simulink model "My_gfm_battery_sil_x"  (R2018b)
settings: Solver=ode45  StartTime=0.0  StopTime=10  MaxStep=1e-4  RelTol=1e-3
PreLoadFcn:
  | modelDir = fileparts(get_param(bdroot,'FileName'));
  | 
  | load_system(fullfile(modelDir,'controls_element_lib.slx'));
  | load_system(fullfile(modelDir,'test_sequence_lib.slx'));
InitFcn:
  | close all;
  | clear all;
  | clc;
  | 
  | % frequency nominals
  | F_NOM = 60;
  | W_NOM = 2 * pi * F_NOM;
  | 
  | % base values relative to inverter
  | % --------------------------------
  | VLL_INV_NOM = 480;
  | P_INV_NOM = 1e6;
  | Q_INV_NOM = 0.5e6;
  | S_INV_NOM = sqrt(P_INV_NOM^2 + Q_INV_NOM^2);
  | 
  | I_INV_BASE = S_INV_NOM/(sqrt(3)*VLL_INV_NOM);
  | Z_INV_BASE = VLL_INV_NOM^2/S_INV_NOM;
  | L_INV_BASE = Z_INV_BASE / W_NOM;
  | C_INV_BASE = 1 / (Z_INV_BASE * W_NOM);
  | 
  | % nominal ratings for power system model
  | % --------------------------------------
  | INVERTER_COUNT = 100;
  | 
  | VLV_NOM = VLL_INV_NOM;
  | VMV_NOM = 35e3;
  | VHV_NOM = 230e3;
  | S_PLANT = INVERTER_COUNT * S_INV_NOM;
  | 
  | N_GSU = VHV_NOM/VMV_NOM;
  | N_MVT = VMV_NOM/VLV_NOM;
  | 
  | I_LV_BASE = S_PLANT/(sqrt(3)*VLV_NOM);
  | I_MV_BASE = S_PLANT/(sqrt(3)*VMV_NOM);
  | I_HV_BASE = S_PLANT/(sqrt(3)*VHV_NOM);
  | 
  | Z_LV_BASE = VLV_NOM^2/S_PLANT;
  | Z_MV_BASE = VMV_NOM^2/S_PLANT;
  | Z_HV_BASE = VHV_NOM^2/S_PLANT;
  | 
  | L_LV_BASE = Z_LV_BASE / W_NOM;
  | L_MV_BASE = Z_MV_BASE / W_NOM;
  | L_HV_BASE = Z_HV_BASE / W_NOM;
  | C_LV_BASE = 1 / (Z_LV_BASE * W_NOM);
  | C_MV_BASE = 1 / (Z_MV_BASE * W_NOM);
  | C_HV_BASE = 1 / (Z_HV_BASE * W_NOM);
undefined symbols (not defined in the file): j
libraries: controls_element_lib x19, simulink x19, test_sequence_lib x12
(part 1 of 4)
settings Model: SimulationMode=accelerator  Creator=HussamAlatrash  LastModifiedBy=ahhei
settings DataIOCC: ReturnWorkspaceOutputs=on
settings OptimizationCC: EfficientMapNaN2IntZero=off
settings DebuggingCC: UnconnectedInputMsg=none  UnconnectedOutputMsg=none  UnconnectedLineMsg=none
settings HardwareCC: TargetBitPerPointer=64  TargetBitPerSizeT=64  TargetBitPerPtrDiffT=64  TargetLongLongMode=on  TargetIntDivRoundTo=Zero  TargetEndianess=LittleEndian  TargetWordSize=64  TargetHWDeviceType=MATLAB Host  ProdEqTarget=off
settings ModelReferenceCC: EnableRefExpFcnMdlSchedulingChecks=off
settings CodeAppCC: MaxIdLength=128
settings GRTTargetCC: TargetLangStandard=C89/C90 (ANSI)  CombineOutputUpdateFcns=off  GRTInterface=on

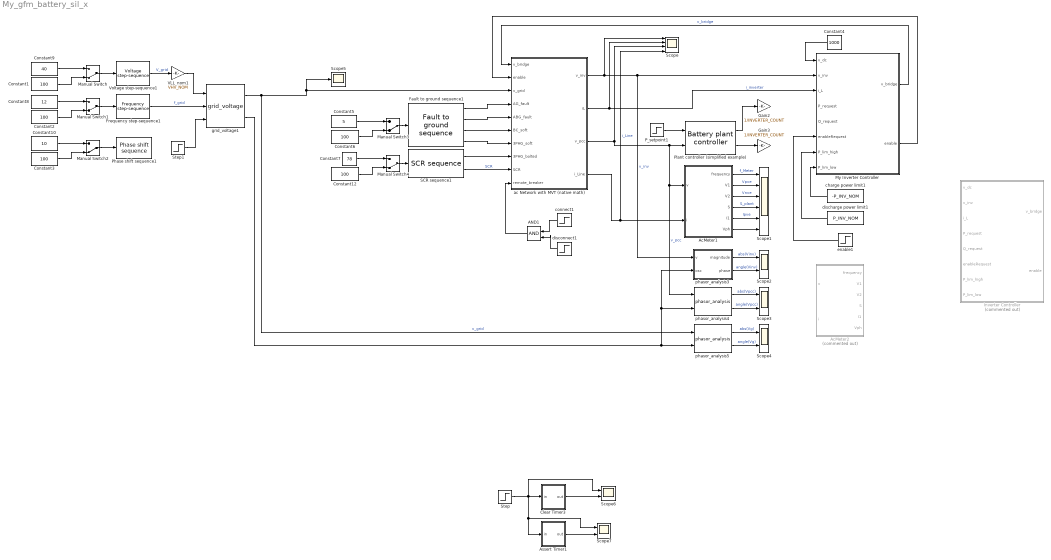
== system My_gfm_battery_sil_x ==
  " Inverter Controller" : Subsystem  Commented=on
  AND1 : Logic  IconShape=distinctive  AllPortsSameDT=off  OutDataTypeStr=boolean
  AcMeter1 : Subsystem  AncestorBlock=test_sequence_lib/AcMeter  mask{VllRated=VHV_NOM}
      mask prompts: VllRated "Rated line voltage"
  AcMeter2 : Subsystem  Commented=on  AncestorBlock=test_sequence_lib/AcMeter  mask{VllRated=VHV_NOM}
      mask prompts: VllRated "Rated line voltage"
  Assert Timer1 : Subsystem  mask{T_STEP=1e-3, TIMEOUT=3e-3}
      mask prompts: T_STEP "Time step"
  Clear Timer3 : Subsystem  mask{T_STEP=1e-3, TIMEOUT=3e-3, TIMER_INIT=0}
      mask prompts: T_STEP "Time step"; TIMER_INIT "Timer initial value"
  Constant{1..3,6,12} (5 alike) : Constant  Value=100
  Constant10 : Constant  Value=10
  Constant4 : Constant  Value=1000
  Constant5 : Constant  Value=5
  Constant7 : Constant  Value=78
  Constant8 : Constant  Value=12
  Constant9 : Constant  Value=40
  Fault to ground sequence1 : test_sequence_lib/Fault to ground sequence  SystemSampleTime=-1
  Frequency step-sequence1 : test_sequence_lib/Frequency step-sequence  SystemSampleTime=-1
  Gain2 : Gain  Gain=1/INVERTER_COUNT
  Gain3 : Gain  Gain=1/INVERTER_COUNT
  Manual Switch{,1..4} (5 alike) : ManualSwitch  CurrentSetting=0
  "My Inverter Controller " : Subsystem
  P_setpoint1 : Step  Time=4  After=S_PLANT*0.5  SampleTime=0
  Phase shift sequence1 : test_sequence_lib/Phase shift sequence  SystemSampleTime=-1
  Plant controller (simplified example) : controls_element_lib/Battery plant controller  SystemSampleTime=-1
  SCR sequence1 : test_sequence_lib/SCR sequence  SystemSampleTime=-1
  Scope : Scope  NumInputPorts=4
  Scope1 : Scope  NumInputPorts=6
  Scope{2..4,6..7} (5 alike) : Scope  NumInputPorts=2
  Scope5 : Scope
  Step : Step  Before=1  After=0  SampleTime=0
  Step1 : Step  Time=6  After=10*pi/180  SampleTime=0
  VLL_nom1 : Gain  Gain=VHV_NOM
  Voltage step-sequence1 : test_sequence_lib/Voltage step-sequence  SystemSampleTime=-1
  ac Network with MVT (native math) : Subsystem  AncestorBlock=test_sequence_lib/ac Network with MVT (native math)
  charge power limit1 : Constant  Value=-P_INV_NOM
  connect1 : Step  Time=0  SampleTime=0
  discharge power limit1 : Constant  Value=P_INV_NOM
  disconnect1 : Step  Time=10  Before=1  After=0  SampleTime=0
  enable1 : Step  Time=0.5  SampleTime=0
  grid_voltage1 : test_sequence_lib/grid_voltage  SystemSampleTime=-1
  phasor_analysis3 : Subsystem  AncestorBlock=test_sequence_lib/phasor_analysis
  phasor_analysis4 : test_sequence_lib/phasor_analysis  SystemSampleTime=-1
  phasor_analysis5 : test_sequence_lib/phasor_analysis  SystemSampleTime=-1
  wires:
  Voltage step-sequence1/1 -> VLL_nom1/1  "V_grid"
  Manual Switch/1 -> Voltage step-sequence1/1
  Fault to ground sequence1/2 -> ac Network with MVT (native math)/5(ABG_fault)
  AND1/1 -> ac Network with MVT (native math)/10(remote_breaker)
  Constant4/1 -> "My Inverter Controller "/1(v_dc)
  AcMeter1/3(V2) -> Scope1/3  "Vnve"
  discharge power limit1/1 -> "My Inverter Controller "/7(P_lim_high)
  Fault to ground sequence1/3 -> ac Network with MVT (native math)/6(BC_soft)
  AcMeter1/6(Vph) -> Scope1/6
  "My Inverter Controller "/1(v_bridge) -> ac Network with MVT (native math)/1(v_bridge)  "v_bridge"
  AcMeter1/2(V1) -> Scope1/2  "Vpve"
  Plant controller (simplified example)/1 -> Gain2/1
  ac Network with MVT (native math)/1(v_inv) -> phasor_analysis3/1(v), "My Inverter Controller "/2(v_inv), Scope/1  "v_inv"
  P_setpoint1/1 -> Plant controller (simplified example)/1
  phasor_analysis5/1 -> Scope4/1  "abs(Vg)"
  AcMeter1/5(I1) -> Scope1/5  "Ipve"
  Plant controller (simplified example)/2 -> Gain3/1
  grid_voltage1/1 -> phasor_analysis5/1, Scope5/1, ac Network with MVT (native math)/3(v_grid)  "v_grid"
  SCR sequence1/1 -> ac Network with MVT (native math)/8(3PHG_bolted)
  phasor_analysis3/1(magnitude) -> Scope2/1  "abs(Vinv)"
  AcMeter1/4(S) -> Scope1/4  "S_plant"
  ac Network with MVT (native math)/4(i_Line) -> Scope/4, AcMeter1/2(i)  "i_Line"
  AcMeter1/1(frequency) -> Scope1/1  "f_Meter"
  VLL_nom1/1 -> grid_voltage1/1
  phasor_analysis3/2(phase) -> Scope2/2  "angle(Vinv)"
  SCR sequence1/2 -> ac Network with MVT (native math)/9(SCR)  "SCR"
  ac Network with MVT (native math)/2(iL) -> "My Inverter Controller "/3(i_L), Scope/2  "i_inverter"
  disconnect1/1 -> AND1/2
  Fault to ground sequence1/4 -> ac Network with MVT (native math)/7(3PHG_soft)
  ac Network with MVT (native math)/3(v_pcc) -> Plant controller (simplified example)/2, phasor_analysis4/1, AcMeter1/1(v), Scope/3  "v_pcc"
  charge power limit1/1 -> "My Inverter Controller "/8(P_lim_low)
  "My Inverter Controller "/2(enable) -> ac Network with MVT (native math)/2(enable)
  Frequency step-sequence1/1 -> grid_voltage1/2  "f_grid"
  Fault to ground sequence1/1 -> ac Network with MVT (native math)/4(AG_fault)
  grid_voltage1/2 -> phasor_analysis4/2, phasor_analysis3/2(osc), phasor_analysis5/2
  phasor_analysis5/2 -> Scope4/2  "angle(Vg)"
  enable1/1 -> "My Inverter Controller "/6(enableRequest)
  connect1/1 -> AND1/1
  Constant9/1 -> Manual Switch/1
  Constant1/1 -> Manual Switch/2
  Constant2/1 -> Manual Switch1/2
  Manual Switch1/1 -> Frequency step-sequence1/1
  Constant8/1 -> Manual Switch1/1
  Manual Switch2/1 -> Phase shift sequence1/1
  Constant3/1 -> Manual Switch2/2
  Constant10/1 -> Manual Switch2/1
  Constant6/1 -> Manual Switch3/2
  Constant5/1 -> Manual Switch3/1
  Manual Switch3/1 -> Fault to ground sequence1/1
  Constant7/1 -> Manual Switch4/1
  Constant12/1 -> Manual Switch4/2
  Manual Switch4/1 -> SCR sequence1/1
  phasor_analysis4/1 -> Scope3/1  "abs(Vpcc)"
  phasor_analysis4/2 -> Scope3/2  "angle(Vpcc)"
  Step/1 -> Scope7/1, Assert Timer1/1(in), Scope6/1, Clear Timer3/1(in)
  Clear Timer3/1(out) -> Scope6/2
  Assert Timer1/1(out) -> Scope7/2
  Step1/1 -> grid_voltage1/3

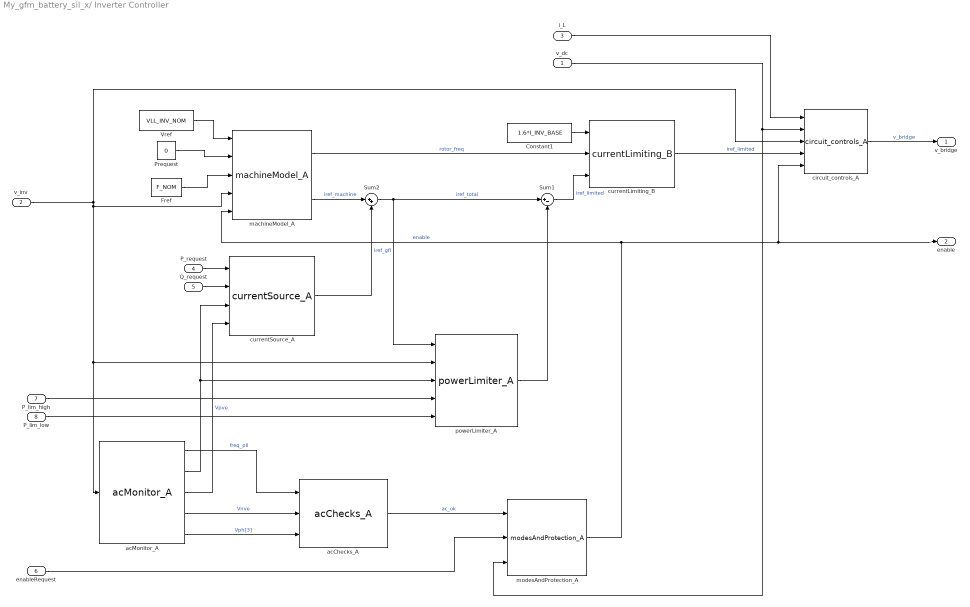
== system My_gfm_battery_sil_x/ Inverter Controller ==
  v_dc : Inport
  v_inv : Inport  Port=2
  i_L : Inport  Port=3
  P_request : Inport  Port=4
  Q_request : Inport  Port=5
  enableRequest : Inport  Port=6
  P_lim_high : Inport  Port=7
  P_lim_low : Inport  Port=8
  Constant1 : Constant  Value=1.6*I_INV_BASE
  Fref : Constant  Value=F_NOM
  Prequest : Constant  Value=0
  Sum1 : Sum  Inputs=|+-
  Sum2 : Sum  Inputs=|++
  Vref : Constant  Value=VLL_INV_NOM
  acChecks_A : controls_element_lib/acChecks_A  VllRated=VLL_INV_NOM  nominalFrequency=F_NOM  tRequalify=2  T_CNTL=1e-3
  "acMonitor_A " : controls_element_lib/acMonitor_A  VllRated=VLL_INV_NOM  nominalFrequency=F_NOM
  circuit_controls_A : controls_element_lib/circuit_controls_A  SystemSampleTime=-1
  currentLimiting_B : controls_element_lib/currentLimiting_B  IRated=I_INV_BASE  peakSoftLimit=2.6  peakHardLimit=3.6
  currentSource_A : controls_element_lib/currentSource_A  VllRated=VLL_INV_NOM  SRated=S_INV_NOM  nominalFrequency=F_NOM  Plimit=P_INV_NOM/S_INV_NOM  Qlimit=Q_INV_NOM/S_INV_NOM
  machineModel_A : controls_element_lib/machineModel_A  SRated=S_INV_NOM  VllRated=VLL_INV_NOM  nominalFrequency=F_NOM  inertialConstant=2.5  kDroop=1  kDamper=2  Xs=0.3  rs=0.08  Qlimit=0.5  wExciter=10
  modesAndProtection_A : controls_element_lib/modesAndProtection_A  dcOvervotlageThreshold=1800  dcUndervotlageThreshold=700  dcTripClearTimeout=0.2
  powerLimiter_A : controls_element_lib/powerLimiter_A  VllRated=VLL_INV_NOM  nominalFrequency=F_NOM  wPowerLimiter=3
  v_bridge : Outport  VectorParamsAs1DForOutWhenUnconnected=on
  enable : Outport  Port=2  VectorParamsAs1DForOutWhenUnconnected=on
  wires:
  Vref/1 -> machineModel_A/1
  Prequest/1 -> machineModel_A/2
  Fref/1 -> machineModel_A/3
  machineModel_A/2 -> Sum2/1  "iref_machine"
  "acMonitor_A "/2 -> currentSource_A/3, powerLimiter_A/3
  Sum1/1 -> currentLimiting_B/3  "iref_limited"
  currentSource_A/1 -> Sum2/2  "iref_gfl"
  Sum2/1 -> Sum1/1, powerLimiter_A/1  "iref_total"
  "acMonitor_A "/3 -> currentSource_A/4  "Vpve"
  Q_request/1 -> currentSource_A/2
  P_request/1 -> currentSource_A/1
  enableRequest/1 -> modesAndProtection_A/2
  modesAndProtection_A/1 -> circuit_controls_A/5, enable/1, machineModel_A/5  "enable"
  "acMonitor_A "/5 -> acChecks_A/3  "Vph[3]"
  acChecks_A/1 -> modesAndProtection_A/1  "ac_ok"
  Constant1/1 -> currentLimiting_B/1
  "acMonitor_A "/1 -> acChecks_A/1  "freq_pll"
  "acMonitor_A "/4 -> acChecks_A/2  "Vnve"
  P_lim_low/1 -> powerLimiter_A/5
  P_lim_high/1 -> powerLimiter_A/4
  powerLimiter_A/1 -> Sum1/2
  v_dc/1 -> circuit_controls_A/2, modesAndProtection_A/3
  circuit_controls_A/1 -> v_bridge/1  "v_bridge"
  machineModel_A/1 -> currentLimiting_B/2  "rotor_freq"
  i_L/1 -> circuit_controls_A/1
  v_inv/1 -> "acMonitor_A "/1, powerLimiter_A/2, machineModel_A/4, circuit_controls_A/3
  currentLimiting_B/1 -> circuit_controls_A/4  "iref_limited"

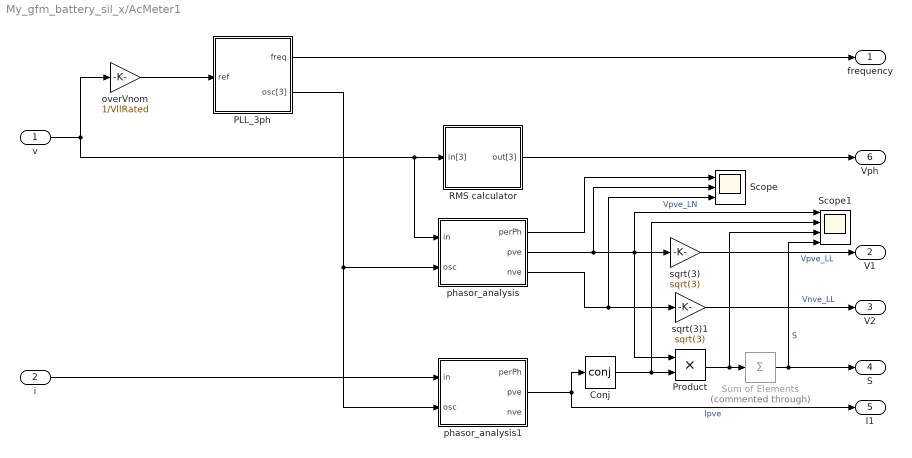
== system My_gfm_battery_sil_x/AcMeter1 ==
  v : Inport
  i : Inport  Port=2
  Conj : Math  Operator=conj  SaturateOnIntegerOverflow=on
  PLL_3ph : Subsystem
  Product : Product
  RMS calculator : Subsystem
  Scope : Scope  NumInputPorts=3
  Scope1 : Scope  NumInputPorts=4
  Sum of Elements : Sum  Commented=through  Inputs=+
  overVnom : Gain  Gain=1/VllRated
  phasor_analysis : Subsystem
  phasor_analysis1 : Subsystem  AncestorBlock=test_sequence_lib/AcMeter/phasor_analysis
  sqrt(3) : Gain  Gain=sqrt(3)
  sqrt(3)1 : Gain  Gain=sqrt(3)
  frequency : Outport  VectorParamsAs1DForOutWhenUnconnected=on
  V1 : Outport  Port=2  VectorParamsAs1DForOutWhenUnconnected=on
  V2 : Outport  Port=3  VectorParamsAs1DForOutWhenUnconnected=on
  S : Outport  Port=4  VectorParamsAs1DForOutWhenUnconnected=on
  I1 : Outport  Port=5  VectorParamsAs1DForOutWhenUnconnected=on
  Vph : Outport  Port=6  VectorParamsAs1DForOutWhenUnconnected=on
  wires:
  RMS calculator/1(out[3]) -> Vph/1
  PLL_3ph/2(osc[3]) -> phasor_analysis/2(osc), phasor_analysis1/2(osc)
  phasor_analysis/1(perPh) -> Scope/1
  Sum of Elements/1 -> Scope1/4, S/1  "S"
  v/1 -> RMS calculator/1(in[3]), phasor_analysis/1(in), overVnom/1
  PLL_3ph/1(freq) -> frequency/1
  overVnom/1 -> PLL_3ph/1(ref)
  Conj/1 -> Scope1/2, Product/2
  Product/1 -> Scope1/3, Sum of Elements/1
  phasor_analysis/2(pve) -> Scope/2, Scope1/1, Product/1, sqrt(3)/1  "Vpve_LN"
  phasor_analysis/3(nve) -> Scope/3, sqrt(3)1/1
  phasor_analysis1/2(pve) -> I1/1, Conj/1  "Ipve"
  sqrt(3)1/1 -> V2/1  "Vnve_LL"
  i/1 -> phasor_analysis1/1(in)
  sqrt(3)/1 -> V1/1  "Vpve_LL"

== system My_gfm_battery_sil_x/AcMeter2 ==
  v : Inport
  i : Inport  Port=2
  Conj : Math  Operator=conj  SaturateOnIntegerOverflow=on
  PLL_3ph : Subsystem
  Product : Product
  RMS calculator : Subsystem
  Scope : Scope  NumInputPorts=3
  Scope1 : Scope  NumInputPorts=4
  Sum of Elements : Sum  Inputs=+
  overVnom : Gain  Gain=1/VllRated
  phasor_analysis : Subsystem
  phasor_analysis1 : Subsystem  AncestorBlock=test_sequence_lib/AcMeter/phasor_analysis
  sqrt(3) : Gain  Gain=sqrt(3)
  sqrt(3)1 : Gain  Gain=sqrt(3)
  frequency : Outport  VectorParamsAs1DForOutWhenUnconnected=on
  V1 : Outport  Port=2  VectorParamsAs1DForOutWhenUnconnected=on
  V2 : Outport  Port=3  VectorParamsAs1DForOutWhenUnconnected=on
  S : Outport  Port=4  VectorParamsAs1DForOutWhenUnconnected=on
  I1 : Outport  Port=5  VectorParamsAs1DForOutWhenUnconnected=on
  Vph : Outport  Port=6  VectorParamsAs1DForOutWhenUnconnected=on
  wires:
  RMS calculator/1(out[3]) -> Vph/1
  PLL_3ph/2(osc[3]) -> phasor_analysis/2(osc), phasor_analysis1/2(osc)
  phasor_analysis/1(perPh) -> Scope/1, Product/1, Scope1/1
  Sum of Elements/1 -> Scope1/4, S/1  "S"
  v/1 -> RMS calculator/1(in[3]), phasor_analysis/1(in), overVnom/1
  PLL_3ph/1(freq) -> frequency/1
  phasor_analysis1/1(perPh) -> Conj/1
  overVnom/1 -> PLL_3ph/1(ref)
  Conj/1 -> Scope1/2, Product/2
  Product/1 -> Scope1/3, Sum of Elements/1
  phasor_analysis/2(pve) -> Scope/2, sqrt(3)/1  "Vpve_LN"
  phasor_analysis/3(nve) -> Scope/3, sqrt(3)1/1
  phasor_analysis1/2(pve) -> I1/1  "Ipve"
  sqrt(3)1/1 -> V2/1  "Vnve_LL"
  i/1 -> phasor_analysis1/1(in)
  sqrt(3)/1 -> V1/1  "Vpve_LL"

== system My_gfm_battery_sil_x/Assert Timer1 ==
  in : Inport
  Constant : Constant  Value=T_STEP
  Constant1 : Constant  Value=0
  Constant2 : Constant  Value=TIMEOUT
  Constant3 : Constant  Value=T_STEP
  Gain : Gain  Gain=0
  Min1 : MinMax  Function=max  Inputs=2
  Min2 : MinMax  Inputs=2
  Relational Operator : RelationalOperator  Operator=>  OutDataTypeStr=boolean  RndMeth=Simplest
  Sum1 : Sum  Inputs=|++
  Sum2 : Sum  Inputs=|++
  Switch : Switch  Criteria=u2 > Threshold
  Unit Delay : UnitDelay  SampleTime=T_STEP
  out : Outport  VectorParamsAs1DForOutWhenUnconnected=on
  wires:
  Sum2/1 -> Relational Operator/1, Min2/1
  Sum1/1 -> Min2/2, Relational Operator/2
  Constant/1 -> Sum2/1
  Min2/1 -> Switch/1
  Constant1/1 -> Switch/3
  Unit Delay/1 -> Sum2/2
  in/1 -> Switch/2
  Switch/1 -> Unit Delay/1
  Relational Operator/1 -> out/1
  Min1/1 -> Sum1/1
  Constant2/1 -> Min1/1
  Constant3/1 -> Min1/2, Gain/1
  Gain/1 -> Sum1/2

== system My_gfm_battery_sil_x/Clear Timer3 ==
  note: One sample delay on Rise
  in : Inport
  Constant : Constant  Value=T_STEP
  Constant1 : Constant  Value=0
  Constant2 : Constant  Value=TIMEOUT
  Constant3 : Constant  Value=T_STEP
  Min1 : MinMax  Function=max  Inputs=2
  Min2 : MinMax  Function=max  Inputs=2
  Relational Operator : RelationalOperator  Operator=>  OutDataTypeStr=boolean  RndMeth=Simplest
  Sum1 : Sum  Inputs=|++
  Sum2 : Sum  Inputs=|-+
  Switch : Switch  Criteria=u2 > Threshold
  Unit Delay : UnitDelay  InitialCondition=TIMER_INIT  SampleTime=T_STEP
  out : Outport  VectorParamsAs1DForOutWhenUnconnected=on
  wires:
  Sum1/1 -> Switch/1
  Sum2/1 -> Relational Operator/1, Min2/1
  Constant/1 -> Sum2/1
  Min2/1 -> Switch/3
  Constant1/1 -> Min2/2, Relational Operator/2
  Unit Delay/1 -> Sum2/2
  in/1 -> Switch/2
  Switch/1 -> Unit Delay/1
  Relational Operator/1 -> out/1
  Constant2/1 -> Min1/1
  Constant3/1 -> Min1/2, Sum1/2
  Min1/1 -> Sum1/1

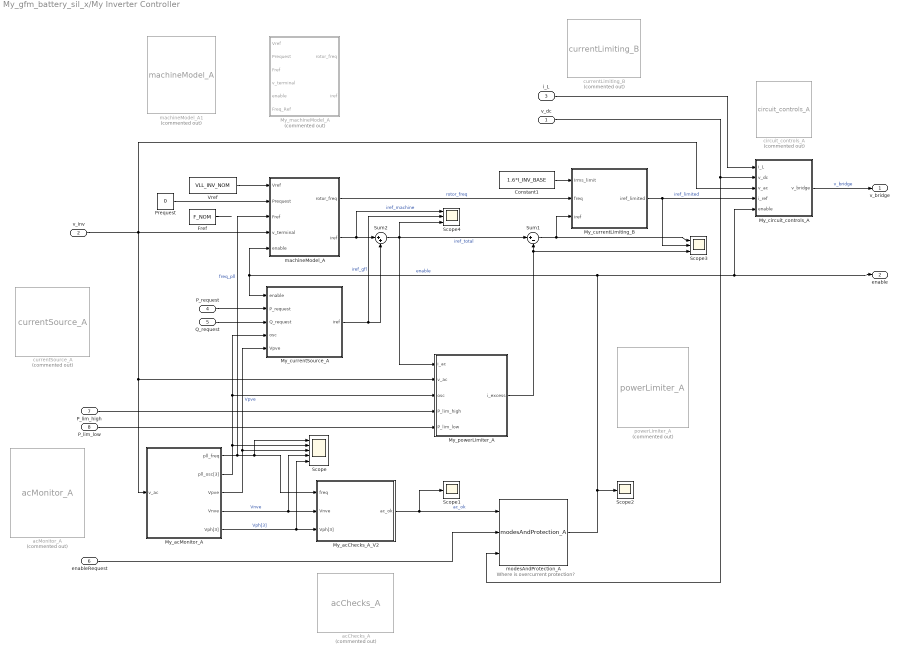
== system My_gfm_battery_sil_x/My Inverter Controller  ==
  note: Where is overcurrent protection?
  v_dc : Inport
  v_inv : Inport  Port=2
  i_L : Inport  Port=3
  P_request : Inport  Port=4
  Q_request : Inport  Port=5
  enableRequest : Inport  Port=6
  P_lim_high : Inport  Port=7
  P_lim_low : Inport  Port=8
  Constant1 : Constant  Value=1.6*I_INV_BASE
  Fref : Constant  Value=F_NOM
  My_acChecks_A_V2 : Subsystem  AncestorBlock=controls_element_lib/acChecks_A  mask{VllRated=VLL_INV_NOM, NominalFrequency=F_NOM, Ts=1e-3, Time1=2, Time2=0, VHi=1.15, VLo=0.85, FHi=62, FLo=58, VNeg=0.2, Time3=0, OV3=1.3, OV3_Time=0.02, OV3_en=1, OV2=1.25, OV2_Time=2, OV2_en=1, OV1=1.2, OV1_Time=20, OV1_en=1, UV1=0.81, UV1_Time=15, UV1_en=1, UV2=0.5, UV2_Time=5, UV2_en=1, UV3=0.2, UV3_Time=1, UV3_en=1, OF3=70, OF3_Time=0.2, OF3_en=1, OF2=65, OF2_Time=10, OF2_en=1, OF1=63, OF1_Time=30, OF1_en=1, UF1=56, UF1_Time=30, UF1_en=1, UF2=55, UF2_Time=10, UF2_en=1, UF3=50, UF3_Time=0.2, UF3_en=1}
      mask prompts: VllRated "Rated Line-to-Line Voltage (V)"; NominalFrequency "Nominal Line Frequency (Hz)"; Ts "Operating Sample Time (sec)"; Time1 "Connection Time (sec)"; Time2 "Connection Out-of-Condition Delay (sec)"; VHi "High Voltage Threshold (pu)"; VLo "Low Voltage Threshold (pu)"; FHi "High Frequency Threshold (Hz)"; FLo "Low Frequency Threshold (Hz)"; VNeg "Negative Sequence Voltage Threshold (pu)"; Time3 "Trip Out-of-Condition Delay (sec)"; OV3 "OV PickUp 3 (pu)"; OV3_Time "OV Time 3 (sec)"; OV3_en "OV Enable 3"; OV2 "OV PickUp 2 (pu)"; OV2_Time "OV Time 2 (sec)"; OV2_en "OV Enable 2"; OV1 "OV PickUp 1 (pu)"; OV1_Time "OV Time 1 (sec)"; OV1_en "OV Enable 1"; UV1 "UV PickUp 1 (pu)"; UV1_Time "UV Time 1 (sec)"; UV1_en "UV Enable 1"; UV2 "UV PickUp 2 (pu)"; UV2_Time "UV Time 2 (sec)"; UV2_en "UV Enable 2"; UV3 "UV PickUp 3 (pu)"; UV3_Time "UV Time 3 (sec)"; UV3_en "UV Enable 3"; OF3 "OF PickUp 3 (Hz)"; OF3_Time "OF Time 3 (pu)"; OF3_en "OF Enable 3"; OF2 "OF PickUp 2 (Hz)"; OF2_Time "OF Time 2 (pu)"; OF2_en "OF Enable 2"; OF1 "OF PickUp 1 (Hz)"; OF1_Time "OF Time 1 (pu)"; OF1_en "OF Enable 1"; UF1 "UF PickUp 1 (Hz)"; UF1_Time "UF Time 1 (sec)"; UF1_en "UF Enable 1"; UF2 "UF PickUp 2 (Hz)"; UF2_Time "UF Time 2 (sec)"; UF2_en "UF Enable 2"; UF3 "UF PickUp 3 (Hz)"; UF3_Time "UF Time 3 (sec)"; UF3_en "UF Enable 3"
      mask DialogControl DescGroupVar Prompt: ACChecks
      mask DialogControl DecsTextVar Prompt: Grid Checks for Connection and Tripping
      mask DialogControl ParameterGroupVar Prompt: General Parameters
      mask DialogControl Container11 Prompt: Connection Settings
      mask DialogControl Container20 Prompt: Thresholds
      mask DialogControl Container3 Prompt: Trip Settings
      mask DialogControl Container12 Prompt: General Parameters
      mask DialogControl Container15 Prompt: Over Voltage Settings
      mask DialogControl Container4 Prompt: Over Voltage
      mask DialogControl Container19 Prompt: Under Voltage Settings
      mask DialogControl Container7 Prompt: Under Voltage
      mask DialogControl Container17 Prompt: Over Frequency Settings
      mask DialogControl Container9 Prompt: Over Frequency
      mask DialogControl Container16 Prompt: Under Frequency Settings
      mask DialogControl Container10 Prompt: Under Frequency
  My_acMonitor_A : Subsystem  AncestorBlock=controls_element_lib/acMonitor_A  mask{VllRated=VLL_INV_NOM, nominalFrequency=F_NOM}
      mask prompts: VllRated "Rated line-to-line voltage (V)"; nominalFrequency "Nominal line frequency (Hz)"
  My_circuit_controls_A : Subsystem  AncestorBlock=controls_element_lib/circuit_controls_A
  My_currentLimiting_B : Subsystem  AncestorBlock=controls_element_lib/currentLimiting_B  mask{IRated=I_INV_BASE, peakSoftLimit=2.6, peakHardLimit=3.6}
      mask prompts: IRated "Rated current (A)"; peakSoftLimit "Soft peak limit (pu)"; peakHardLimit "Hard peak limit (pu)"
  My_currentSource_A : Subsystem  AncestorBlock=controls_element_lib/currentSource_A  mask{VllRated=VLL_INV_NOM, SRated=S_INV_NOM, nominalFrequency=F_NOM, Plimit=P_INV_NOM/S_INV_NOM, Qlimit=Q_INV_NOM/S_INV_NOM}
      mask prompts: VllRated "Rated line-to-line voltage (V)"; SRated "Rated power (VA)"; nominalFrequency "Nominal line frequency (Hz)"; Plimit "Real power request limit (pu)"; Qlimit "Reactive power request limit (pu)"
  My_machineModel_A : Subsystem  Commented=on  AncestorBlock=controls_element_lib/machineModel_A  mask{SRated=S_INV_NOM, VllRated=VLL_INV_NOM, nominalFrequency=F_NOM, inertialConstant=2.5, kDroop=1, kDamper=2, Xs=0.3, rs=0.08, Qlimit=0.5, wExciter=10, FreqFF_Sel=0}
      mask prompts: SRated "Rated power (VA)"; VllRated "Rated Voltage (Volts, line-to-line)"; nominalFrequency "Nominal frequency (Hz)"; inertialConstant "Inertial constant (seconds)"; kDroop "Droop gain (pu/Hz)"; kDamper "Damper gain (pu/Hz)"; Xs "Stator reactance (pu)"; rs "Stator resistance (pu)"; Qlimit "Reactive power request limit (pu)"; wExciter "Exciter Bandwidth (rad)"; FreqFF_Sel "Frequency Feedforward Selector"
  My_powerLimiter_A : Subsystem  AncestorBlock=controls_element_lib/powerLimiter_A  mask{VllRated=VLL_INV_NOM, nominalFrequency=F_NOM, wPowerLimiter=3}
      mask prompts: VllRated "Rated line-to-line voltage (V)"; nominalFrequency "Nominal line frequency (Hz)"; wPowerLimiter "Bandwidth (rad)"
  Prequest : Constant  Value=0
  Scope : Scope  NumInputPorts=5
  Scope1 : Scope
  Scope2 : Scope
  Scope3 : Scope  NumInputPorts=3
  Scope4 : Scope  NumInputPorts=3
  Sum1 : Sum  Inputs=|+-
  Sum2 : Sum  Inputs=|++
  Vref : Constant  Value=VLL_INV_NOM
  acChecks_A : controls_element_lib/acChecks_A  Commented=on  VllRated=VLL_INV_NOM  nominalFrequency=F_NOM  tRequalify=2  T_CNTL=1e-3
  acMonitor_A : controls_element_lib/acMonitor_A  Commented=on  VllRated=VLL_INV_NOM  nominalFrequency=F_NOM
  circuit_controls_A : controls_element_lib/circuit_controls_A  Commented=on  SystemSampleTime=-1
  currentLimiting_B : controls_element_lib/currentLimiting_B  Commented=on  IRated=I_INV_BASE  peakSoftLimit=2.6  peakHardLimit=3.6
  currentSource_A : controls_element_lib/currentSource_A  Commented=on  VllRated=VLL_INV_NOM  SRated=S_INV_NOM  nominalFrequency=F_NOM  Plimit=P_INV_NOM/S_INV_NOM  Qlimit=Q_INV_NOM/S_INV_NOM
  machineModel_A : Subsystem  AncestorBlock=controls_element_lib/machineModel_A  mask{SRated=S_INV_NOM, VllRated=VLL_INV_NOM, nominalFrequency=F_NOM, inertialConstant=2.5, kDroop=1, kDamper=2, Xs=0.3, rs=0.08, Qlimit=0.5, wExciter=10}
      mask prompts: SRated "Rated power (VA)"; VllRated "Rated Voltage (Volts, line-to-line)"; nominalFrequency "Nominal frequency (Hz)"; inertialConstant "Inertial constant (seconds)"; kDroop "Droop gain (pu/Hz)"; kDamper "Damper gain (pu/Hz)"; Xs "Stator reactance (pu)"; rs "Stator resistance (pu)"; Qlimit "Reactive power request limit (pu)"; wExciter "Exciter Bandwidth (rad)"
  machineModel_A1 : controls_element_lib/machineModel_A  Commented=on  SRated=S_INV_NOM  VllRated=VLL_INV_NOM  nominalFrequency=F_NOM  inertialConstant=2.5  kDroop=1  kDamper=2  Xs=0.3  rs=0.08  Qlimit=0.5  wExciter=10
  modesAndProtection_A : controls_element_lib/modesAndProtection_A  dcOvervotlageThreshold=1800  dcUndervotlageThreshold=700  dcTripClearTimeout=0.2
  powerLimiter_A : controls_element_lib/powerLimiter_A  Commented=on  VllRated=VLL_INV_NOM  nominalFrequency=F_NOM  wPowerLimiter=3
  v_bridge : Outport  VectorParamsAs1DForOutWhenUnconnected=on
  enable : Outport  Port=2  VectorParamsAs1DForOutWhenUnconnected=on
  wires:
  Vref/1 -> machineModel_A/1(Vref)
  Prequest/1 -> machineModel_A/2(Prequest)
  machineModel_A/2(iref) -> Scope4/1, Sum2/1  "iref_machine"
  My_acMonitor_A/2(pll_osc[3]) -> Scope/2, My_currentSource_A/4(osc), My_powerLimiter_A/3(osc)
  My_currentLimiting_B/1(iref_limited) -> My_circuit_controls_A/4(i_ref), Scope3/2  "iref_limited"
  My_currentSource_A/1(iref) -> Sum2/2, Scope4/2  "iref_gfl"
  Sum2/1 -> Sum1/1, Scope4/3, My_powerLimiter_A/1(i_ac)  "iref_total"
  My_acMonitor_A/3(Vpve) -> My_currentSource_A/5(Vpve), Scope/3  "Vpve"
  Q_request/1 -> My_currentSource_A/3(Q_request)
  P_request/1 -> My_currentSource_A/2(P_request)
  enableRequest/1 -> modesAndProtection_A/2
  modesAndProtection_A/1 -> Scope2/1, machineModel_A/5(enable), My_currentSource_A/1(enable), My_circuit_controls_A/5(enable), enable/1  "enable"
  My_acMonitor_A/5(Vph[3]) -> My_acChecks_A_V2/3(Vph[3]), Scope/5  "Vph[3]"
  My_acChecks_A_V2/1(ac_ok) -> Scope1/1, modesAndProtection_A/1  "ac_ok"
  Constant1/1 -> My_currentLimiting_B/1(Irms_limit)
  My_acMonitor_A/1(pll_freq) -> machineModel_A/3(Fref), My_acChecks_A_V2/1(freq), Scope/1  "freq_pll"
  My_acMonitor_A/4(Vnve) -> My_acChecks_A_V2/2(Vnve), Scope/4  "Vnve"
  P_lim_low/1 -> My_powerLimiter_A/5(P_lim_low)
  P_lim_high/1 -> My_powerLimiter_A/4(P_lim_high)
  My_powerLimiter_A/1(i_excess) -> Sum1/2, Scope3/3
  Sum1/1 -> My_currentLimiting_B/3(iref), Scope3/1
  v_dc/1 -> My_circuit_controls_A/2(v_dc), modesAndProtection_A/3
  My_circuit_controls_A/1(v_bridge) -> v_bridge/1  "v_bridge"
  machineModel_A/1(rotor_freq) -> My_currentLimiting_B/2(freq)  "rotor_freq"
  i_L/1 -> My_circuit_controls_A/1(i_L)
  v_inv/1 -> My_acMonitor_A/1(v_ac), My_powerLimiter_A/2(v_ac), machineModel_A/4(v_terminal), My_circuit_controls_A/3(v_ac)
  Fref/1 -> ?

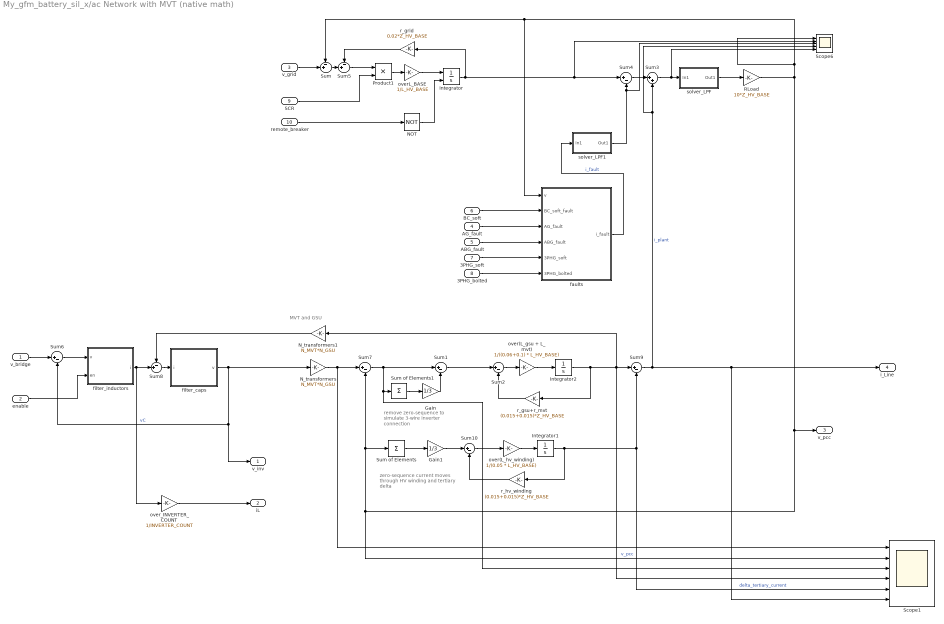
== system My_gfm_battery_sil_x/ac Network with MVT (native math) ==
  note: zero-sequence current moves through HV winding and tertiary delta
  note: remove zero-sequence to simulate 3-wire inverter connection
  note: MVT and GSU
  v_bridge : Inport
  enable : Inport  Port=2
  v_grid : Inport  Port=3
  AG_fault : Inport  Port=4
  ABG_fault : Inport  Port=5
  BC_soft : Inport  Port=6
  3PHG_soft : Inport  Port=7
  3PHG_bolted : Inport  Port=8
  SCR : Inport  Port=9
  remote_breaker : Inport  Port=10
  Gain : Gain  Gain=1/3
  Gain1 : Gain  Gain=1/3
  Integrator : Integrator  ExternalReset=level
  Integrator1 : Integrator
  Integrator2 : Integrator
  NOT : Logic  Operator=NOT  IconShape=distinctive  AllPortsSameDT=off  OutDataTypeStr=boolean
  N_transformers : Gain  Gain=N_MVT*N_GSU
  N_transformers1 : Gain  Gain=N_MVT*N_GSU
  Product1 : Product
  RLoad : Gain  Gain=10*Z_HV_BASE
  Scope1 : Scope  NumInputPorts=6
  Scope6 : Scope  NumInputPorts=5
  Sum : Sum  Inputs=-+|
  Sum of Elements : Sum  Inputs=+
  Sum of Elements1 : Sum  Inputs=+
  Sum{1..2,4,6..7,9..10} (7 alike) : Sum  Inputs=|+-
  Sum3 : Sum  Inputs=|++
  Sum5 : Sum  Inputs=-+|
  Sum8 : Sum  Inputs=-+|
  faults : Subsystem
  filter_caps : Subsystem
  filter_inductors : Subsystem
  over(L_gsu + L_mvt) : Gain  Gain=1/((0.06+0.1) * L_HV_BASE)
  over(L_hv_winding) : Gain  Gain=1/(0.05 * L_HV_BASE)
  overL_BASE : Gain  Gain=1/L_HV_BASE
  over_INVERTER_COUNT : Gain  Gain=1/INVERTER_COUNT
  r_grid : Gain  Gain=0.02*Z_HV_BASE
  r_gsu+r_mvt : Gain  Gain=(0.015+0.015)*Z_HV_BASE
  r_hv_winding : Gain  Gain=(0.015+0.015)*Z_HV_BASE
  solver_LPF : Subsystem
  solver_LPF1 : Subsystem
  v_inv : Outport  VectorParamsAs1DForOutWhenUnconnected=on
  iL : Outport  Port=2  VectorParamsAs1DForOutWhenUnconnected=on
  v_pcc : Outport  Port=3  VectorParamsAs1DForOutWhenUnconnected=on
  i_Line : Outport  Port=4  VectorParamsAs1DForOutWhenUnconnected=on
  wires:
  AG_fault/1 -> faults/3(AG_fault)
  ABG_fault/1 -> faults/4(ABG_fault)
  BC_soft/1 -> faults/2(BC_soft_fault)
  Gain1/1 -> Sum10/1
  Sum of Elements/1 -> Gain1/1
  Sum10/1 -> over(L_hv_winding)/1
  r_hv_winding/1 -> Sum10/2
  Integrator1/1 -> r_hv_winding/1, Scope1/5, Sum9/2  "delta_tertiary_current"
  over(L_hv_winding)/1 -> Integrator1/1
  Sum9/1 -> Scope1/6, i_Line/1, Scope6/4, Sum3/2  "i_plant"
  N_transformers1/1 -> Sum8/1
  N_transformers/1 -> Scope1/1, Sum7/1
  over_INVERTER_COUNT/1 -> iL/1
  filter_caps/1(v) -> N_transformers/1, Sum6/2, v_inv/1  "vC"
  Sum8/1 -> filter_caps/1(i)
  filter_inductors/1(i) -> over_INVERTER_COUNT/1, Sum8/2
  enable/1 -> filter_inductors/2(en)
  Sum6/1 -> filter_inductors/1(v)
  r_gsu+r_mvt/1 -> Sum2/2
  Sum1/1 -> Sum2/1
  Gain/1 -> Sum1/2
  Sum of Elements1/1 -> Gain/1
  Sum2/1 -> over(L_gsu + L_mvt)/1
  Sum7/1 -> Sum1/1, Scope1/3, Sum of Elements1/1
  over(L_gsu + L_mvt)/1 -> Integrator2/1
  solver_LPF/1(Out1) -> RLoad/1
  remote_breaker/1 -> NOT/1
  overL_BASE/1 -> Integrator/1
  Integrator/1 -> Scope6/2, Sum4/1, r_grid/1
  solver_LPF1/1(Out1) -> Scope6/3, Sum4/2
  RLoad/1 -> Sum of Elements/1, Sum7/2, Scope1/2, v_pcc/1, Sum/1, faults/1(v), Scope6/1  "v_pcc"
  faults/1(i_fault) -> solver_LPF1/1(In1)  "i_fault"
  3PHG_bolted/1 -> faults/6(3PHG_bolted)
  v_bridge/1 -> Sum6/1
  Product1/1 -> overL_BASE/1
  SCR/1 -> Product1/2
  r_grid/1 -> Sum5/1
  Sum3/1 -> Scope6/5, solver_LPF/1(In1)
  NOT/1 -> Integrator/2
  Sum4/1 -> Sum3/1
  v_grid/1 -> Sum/2
  Sum5/1 -> Product1/1
  Sum/1 -> Sum5/2
  Integrator2/1 -> Scope1/4, Sum9/1, N_transformers1/1, r_gsu+r_mvt/1
  3PHG_soft/1 -> faults/5(3PHG_soft)

== system My_gfm_battery_sil_x/phasor_analysis3 ==
  v : Inport
  osc : Inport  Port=2
  Complex to Magnitude-Angle : ComplexToMagnitudeAngle
  Complex to Real-Imag : ComplexToRealImag
  Conj : Math  Operator=conj  SaturateOnIntegerOverflow=on
  Gain : Gain  Gain=sqrt(2)
  Gain1 : Gain  Gain=1/3
  Gain2 : Gain  Gain=sqrt(3)
  Product3 : Product
  Real-Imag to Complex : RealImagToComplex
  Scope : Scope  NumInputPorts=4
  Sum of Elements1 : Sum  Inputs=+
  Transfer Fcn : TransferFcn  Denominator=[0.01 1]
  Transfer Fcn1 : TransferFcn  Denominator=[0.01 1]
  magnitude : Outport  VectorParamsAs1DForOutWhenUnconnected=on
  phase : Outport  Port=2  VectorParamsAs1DForOutWhenUnconnected=on
  wires:
  Complex to Magnitude-Angle/2 -> phase/1
  Complex to Magnitude-Angle/1 -> magnitude/1
  Gain2/1 -> Complex to Magnitude-Angle/1
  Gain1/1 -> Complex to Real-Imag/1
  Gain/1 -> Scope/2, Product3/2
  Real-Imag to Complex/1 -> Gain2/1
  Conj/1 -> Gain/1
  osc/1 -> Conj/1
  Complex to Real-Imag/1 -> Transfer Fcn/1
  v/1 -> Scope/1, Product3/1
  Complex to Real-Imag/2 -> Transfer Fcn1/1
  Product3/1 -> Scope/3, Sum of Elements1/1
  Transfer Fcn/1 -> Real-Imag to Complex/1
  Sum of Elements1/1 -> Scope/4, Gain1/1
  Transfer Fcn1/1 -> Real-Imag to Complex/2

== system My_gfm_battery_sil_x/AcMeter1/PLL_3ph ==
  ref : Inport
  Complex to Real-Imag : ComplexToRealImag
  Conj : Math  Operator=conj  SaturateOnIntegerOverflow=on
  Constant : Constant  Value=120
  Gain1 : Gain  Gain=1.5
  Gain2 : Gain  Gain=4.5
  Gain3 : Gain  Gain=10e-3
  Integrator : Integrator  LimitOutput=on  UpperSaturationLimit=5  LowerSaturationLimit=-5
  Product : Product
  SOGI : Subsystem  AncestorBlock=controls_module_lib/dcVoltageRegulator_A/SOGI
  Saturation : Saturate  UpperLimit=5  LowerLimit=-5
  Sum : Sum  Inputs=+++
  Sum of Elements : Sum  Inputs=+
  Sum1 : Sum  Inputs=|+-
  Transfer Fcn : TransferFcn  Denominator=[0.02 1]
  f_nom : Constant  Value=60
  oscillator_3ph : Subsystem
  freq : Outport  VectorParamsAs1DForOutWhenUnconnected=on
  osc[3] : Outport  Port=2  VectorParamsAs1DForOutWhenUnconnected=on
  wires:
  Gain1/1 -> Saturation/1
  Conj/1 -> Complex to Real-Imag/1
  ref/1 -> Product/1
  Integrator/1 -> Sum/3, Gain3/1
  Sum1/1 -> Integrator/1
  Complex to Real-Imag/2 -> Product/2
  Gain2/1 -> Sum1/1
  oscillator_3ph/1(osc[3]) -> osc[3]/1, Conj/1
  Sum/1 -> oscillator_3ph/1(f), freq/1  "freq"
  Product/1 -> Sum of Elements/1
  Saturation/1 -> Sum/2
  SOGI/1(notch) -> Gain2/1, Gain1/1  "phase_error"
  Sum of Elements/1 -> Transfer Fcn/1
  Gain3/1 -> Sum1/2
  f_nom/1 -> Sum/1
  Transfer Fcn/1 -> SOGI/1(in)  "phase_error"
  Constant/1 -> SOGI/2(fnom)

== system My_gfm_battery_sil_x/AcMeter1/RMS calculator ==
  in[3] : Inport
  Gain : Gain  Gain=20
  Integrator : Integrator
  Square : Math  Operator=square  SaturateOnIntegerOverflow=on
  Square Root : Sqrt  SaturateOnIntegerOverflow=on
  Sum : Sum  Inputs=|+-
  out[3] : Outport  VectorParamsAs1DForOutWhenUnconnected=on
  wires:
  in[3]/1 -> Square/1
  Square/1 -> Sum/1
  Gain/1 -> Integrator/1
  Square Root/1 -> out[3]/1  "Vph_rms"
  Sum/1 -> Gain/1
  Integrator/1 -> Square Root/1, Sum/2

== system My_gfm_battery_sil_x/AcMeter1/phasor_analysis ==
  in : Inport
  osc : Inport  Port=2
  Conj : Math  Operator=conj  SaturateOnIntegerOverflow=on
  Conj1 : Math  Operator=conj  SaturateOnIntegerOverflow=on
  Demux : Demux  Outputs=3
  Gain1 : Gain  Gain=1/3
  Gain3 : Gain  Gain=1/3
  Mux : Mux  Inputs=3
  Product1 : Product
  Product3 : Product
  Scope : Scope  NumInputPorts=5
  Sum of Elements1 : Sum  Inputs=+
  Sum of Elements2 : Sum  Inputs=+
  complex_LPF1 : Subsystem  mask{wLPF=50}
      mask prompts: wLPF "Bandwidth (rad/sec)"
  complex_LPF2 : test_sequence_lib/AcMeter/phasor_analysis/complex_LPF1  wLPF=50
  sqrt(2) : Gain  Gain=sqrt(2)
  sqrt(2)1 : Gain  Gain=sqrt(2)
  perPh : Outport  VectorParamsAs1DForOutWhenUnconnected=on
  pve : Outport  Port=2  VectorParamsAs1DForOutWhenUnconnected=on
  nve : Outport  Port=3  VectorParamsAs1DForOutWhenUnconnected=on
  wires:
  complex_LPF2/1 -> Sum of Elements2/1
  Product1/1 -> complex_LPF2/1
  complex_LPF1/1(1) -> Scope/4, perPh/1
  Product3/1 -> Sum of Elements1/1, Scope/3, complex_LPF1/1(In1)
  Sum of Elements1/1 -> Scope/5, Gain1/1
  in/1 -> Scope/1, Product3/1, Product1/1
  osc/1 -> Demux/1, Conj/1
  Conj/1 -> sqrt(2)/1
  sqrt(2)/1 -> Scope/2, Product3/2
  Gain1/1 -> pve/1
  Demux/1 -> Mux/1
  Demux/2 -> Mux/3
  Demux/3 -> Mux/2
  Mux/1 -> Conj1/1
  Conj1/1 -> sqrt(2)1/1
  sqrt(2)1/1 -> Product1/2
  Sum of Elements2/1 -> Gain3/1
  Gain3/1 -> nve/1

== system My_gfm_battery_sil_x/AcMeter1/phasor_analysis1 ==
  in : Inport
  osc : Inport  Port=2
  Conj : Math  Operator=conj  SaturateOnIntegerOverflow=on
  Conj1 : Math  Operator=conj  SaturateOnIntegerOverflow=on
  Demux : Demux  Outputs=3
  Gain1 : Gain  Gain=1/3
  Gain3 : Gain  Gain=1/3
  Mux : Mux  Inputs=3
  Product1 : Product
  Product3 : Product
  Sum of Elements1 : Sum  Inputs=+
  Sum of Elements2 : Sum  Inputs=+
  complex_LPF1 : Subsystem  Commented=through  mask{wLPF=50}
      mask prompts: wLPF "Bandwidth (rad/sec)"
  complex_LPF2 : test_sequence_lib/AcMeter/phasor_analysis/complex_LPF1  wLPF=50
  sqrt(2) : Gain  Gain=sqrt(2)
  sqrt(2)1 : Gain  Gain=sqrt(2)
  perPh : Outport  VectorParamsAs1DForOutWhenUnconnected=on
  pve : Outport  Port=2  VectorParamsAs1DForOutWhenUnconnected=on
  nve : Outport  Port=3  VectorParamsAs1DForOutWhenUnconnected=on
  wires:
  complex_LPF2/1 -> Sum of Elements2/1
  Product1/1 -> complex_LPF2/1
  complex_LPF1/1(1) -> perPh/1, Sum of Elements1/1
  Product3/1 -> complex_LPF1/1(In1)
  Sum of Elements1/1 -> Gain1/1
  in/1 -> Product3/1, Product1/1
  osc/1 -> Demux/1, Conj/1
  Conj/1 -> sqrt(2)/1
  sqrt(2)/1 -> Product3/2
  Gain1/1 -> pve/1
  Demux/1 -> Mux/1
  Demux/2 -> Mux/3
  Demux/3 -> Mux/2
  Mux/1 -> Conj1/1
  Conj1/1 -> sqrt(2)1/1
  sqrt(2)1/1 -> Product1/2
  Sum of Elements2/1 -> Gain3/1
  Gain3/1 -> nve/1

== system My_gfm_battery_sil_x/AcMeter2/PLL_3ph ==
  ref : Inport
  Complex to Real-Imag : ComplexToRealImag
  Conj : Math  Operator=conj  SaturateOnIntegerOverflow=on
  Constant : Constant  Value=120
  Gain1 : Gain  Gain=1.5
  Gain2 : Gain  Gain=4.5
  Gain3 : Gain  Gain=10e-3
  Integrator : Integrator  LimitOutput=on  UpperSaturationLimit=5  LowerSaturationLimit=-5
  Product : Product
  SOGI : Subsystem  AncestorBlock=controls_module_lib/dcVoltageRegulator_A/SOGI
  Saturation : Saturate  UpperLimit=5  LowerLimit=-5
  Sum : Sum  Inputs=+++
  Sum of Elements : Sum  Inputs=+
  Sum1 : Sum  Inputs=|+-
  Transfer Fcn : TransferFcn  Denominator=[0.02 1]
  f_nom : Constant  Value=60
  oscillator_3ph : Subsystem
  freq : Outport  VectorParamsAs1DForOutWhenUnconnected=on
  osc[3] : Outport  Port=2  VectorParamsAs1DForOutWhenUnconnected=on
  wires:
  Gain1/1 -> Saturation/1
  Conj/1 -> Complex to Real-Imag/1
  ref/1 -> Product/1
  Integrator/1 -> Sum/3, Gain3/1
  Sum1/1 -> Integrator/1
  Complex to Real-Imag/2 -> Product/2
  Gain2/1 -> Sum1/1
  oscillator_3ph/1(osc[3]) -> osc[3]/1, Conj/1
  Sum/1 -> oscillator_3ph/1(f), freq/1  "freq"
  Product/1 -> Sum of Elements/1
  Saturation/1 -> Sum/2
  SOGI/1(notch) -> Gain2/1, Gain1/1  "phase_error"
  Sum of Elements/1 -> Transfer Fcn/1
  Gain3/1 -> Sum1/2
  f_nom/1 -> Sum/1
  Transfer Fcn/1 -> SOGI/1(in)  "phase_error"
  Constant/1 -> SOGI/2(fnom)

== system My_gfm_battery_sil_x/AcMeter2/RMS calculator ==
  in[3] : Inport
  Gain : Gain  Gain=20
  Integrator : Integrator
  Square : Math  Operator=square  SaturateOnIntegerOverflow=on
  Square Root : Sqrt  SaturateOnIntegerOverflow=on
  Sum : Sum  Inputs=|+-
  out[3] : Outport  VectorParamsAs1DForOutWhenUnconnected=on
  wires:
  in[3]/1 -> Square/1
  Square/1 -> Sum/1
  Gain/1 -> Integrator/1
  Square Root/1 -> out[3]/1  "Vph_rms"
  Sum/1 -> Gain/1
  Integrator/1 -> Square Root/1, Sum/2

== system My_gfm_battery_sil_x/AcMeter2/phasor_analysis ==
  in : Inport
  osc : Inport  Port=2
  Conj : Math  Operator=conj  SaturateOnIntegerOverflow=on
  Conj1 : Math  Operator=conj  SaturateOnIntegerOverflow=on
  Demux : Demux  Outputs=3
  Gain1 : Gain  Gain=1/3
  Gain3 : Gain  Gain=1/3
  Mux : Mux  Inputs=3
  Product1 : Product
  Product3 : Product
  Scope : Scope  NumInputPorts=5
  Sum of Elements1 : Sum  Inputs=+
  Sum of Elements2 : Sum  Inputs=+
  complex_LPF1 : Subsystem  mask{wLPF=50}
      mask prompts: wLPF "Bandwidth (rad/sec)"
  complex_LPF2 : test_sequence_lib/AcMeter/phasor_analysis/complex_LPF1  wLPF=50
  sqrt(2) : Gain  Gain=sqrt(2)
  sqrt(2)1 : Gain  Gain=sqrt(2)
  perPh : Outport  VectorParamsAs1DForOutWhenUnconnected=on
  pve : Outport  Port=2  VectorParamsAs1DForOutWhenUnconnected=on
  nve : Outport  Port=3  VectorParamsAs1DForOutWhenUnconnected=on
  wires:
  complex_LPF2/1 -> Sum of Elements2/1
  Product1/1 -> complex_LPF2/1
  complex_LPF1/1(1) -> Scope/4, perPh/1
  Product3/1 -> Sum of Elements1/1, Scope/3, complex_LPF1/1(In1)
  Sum of Elements1/1 -> Scope/5, Gain1/1
  in/1 -> Scope/1, Product3/1, Product1/1
  osc/1 -> Demux/1, Conj/1
  Conj/1 -> sqrt(2)/1
  sqrt(2)/1 -> Scope/2, Product3/2
  Gain1/1 -> pve/1
  Demux/1 -> Mux/1
  Demux/2 -> Mux/3
  Demux/3 -> Mux/2
  Mux/1 -> Conj1/1
  Conj1/1 -> sqrt(2)1/1
  sqrt(2)1/1 -> Product1/2
  Sum of Elements2/1 -> Gain3/1
  Gain3/1 -> nve/1

== system My_gfm_battery_sil_x/AcMeter2/phasor_analysis1 ==
  in : Inport
  osc : Inport  Port=2
  Conj : Math  Operator=conj  SaturateOnIntegerOverflow=on
  Conj1 : Math  Operator=conj  SaturateOnIntegerOverflow=on
  Demux : Demux  Outputs=3
  Gain1 : Gain  Gain=1/3
  Gain3 : Gain  Gain=1/3
  Mux : Mux  Inputs=3
  Product1 : Product
  Product3 : Product
  Sum of Elements1 : Sum  Inputs=+
  Sum of Elements2 : Sum  Inputs=+
  complex_LPF1 : Subsystem  mask{wLPF=50}
      mask prompts: wLPF "Bandwidth (rad/sec)"
  complex_LPF2 : test_sequence_lib/AcMeter/phasor_analysis/complex_LPF1  wLPF=50
  sqrt(2) : Gain  Gain=sqrt(2)
  sqrt(2)1 : Gain  Gain=sqrt(2)
  perPh : Outport  VectorParamsAs1DForOutWhenUnconnected=on
  pve : Outport  Port=2  VectorParamsAs1DForOutWhenUnconnected=on
  nve : Outport  Port=3  VectorParamsAs1DForOutWhenUnconnected=on
  wires:
  complex_LPF2/1 -> Sum of Elements2/1
  Product1/1 -> complex_LPF2/1
  complex_LPF1/1(1) -> perPh/1, Sum of Elements1/1
  Product3/1 -> complex_LPF1/1(In1)
  Sum of Elements1/1 -> Gain1/1
  in/1 -> Product3/1, Product1/1
  osc/1 -> Demux/1, Conj/1
  Conj/1 -> sqrt(2)/1
  sqrt(2)/1 -> Product3/2
  Gain1/1 -> pve/1
  Demux/1 -> Mux/1
  Demux/2 -> Mux/3
  Demux/3 -> Mux/2
  Mux/1 -> Conj1/1
  Conj1/1 -> sqrt(2)1/1
  sqrt(2)1/1 -> Product1/2
  Sum of Elements2/1 -> Gain3/1
  Gain3/1 -> nve/1
